simulink model "ElectricVehicleThermalManagementWithHeatPump_2026a_version"  (R2026a)
settings: Solver=VariableStepAuto  StopTime=3600  AbsTol=1e-3
PreLoadFcn:
  | init_nmpc
InitFcn:
  | init_nmpc
model workspace: external: MATLAB File ElectricVehicleThermalManagementWithHeatPumpParameters.m (data not in the file)
values from neighbouring files (symbols this model uses):
  battery_C1_LUT = [1913.6 12447 30609 ... (first row only)    [ElectricVehicleThermalManagementWithHeatPumpParameters.m]
  battery_capacity_LUT = [280.081 276.25 276.392]    [ElectricVehicleThermalManagementWithHeatPumpParameters.m]
  battery_cell_cp = 795    [ElectricVehicleThermalManagementWithHeatPumpParameters.m]
  battery_cell_mass = 2.5    [ElectricVehicleThermalManagementWithHeatPumpParameters.m]
  battery_Em_LUT = [3.4966 3.5057 3.5148 ... (first row only)    [ElectricVehicleThermalManagementWithHeatPumpParameters.m]
  battery_N_cells = 20    [ElectricVehicleThermalManagementWithHeatPumpParameters.m]
  battery_Qe_init = 0    [ElectricVehicleThermalManagementWithHeatPumpParameters.m]
  battery_R0_LUT = [0.0117 0.0085 0.009 ... (first row only)    [ElectricVehicleThermalManagementWithHeatPumpParameters.m]
  battery_R1_LUT = [0.0109 0.0029 0.0013 ... (first row only)    [ElectricVehicleThermalManagementWithHeatPumpParameters.m]
  battery_SOC_LUT = [0; 0.1; 0.25; 0.5; 0.75; 0.9; 1]    [ElectricVehicleThermalManagementWithHeatPumpParameters.m]
  battery_T_init = -5    [ElectricVehicleThermalManagementWithHeatPumpParameters.m]
  battery_temperature_LUT = [5 20 40]    [ElectricVehicleThermalManagementWithHeatPumpParameters.m]
  cabin_duct_area = 0.04    [ElectricVehicleThermalManagementWithHeatPumpParameters.m]
  cabin_T_init = -5    [ElectricVehicleThermalManagementWithHeatPumpParameters.m]
  chiller_area_primary = 0.43982297150257105    (= 0.439822971503)    [ElectricVehicleThermalManagementWithHeatPumpParameters.m]
  chiller_N_baffles = 3    [ElectricVehicleThermalManagementWithHeatPumpParameters.m]
  chiller_N_tubes = 100    [ElectricVehicleThermalManagementWithHeatPumpParameters.m]
  chiller_tube_D = 0.0035    [ElectricVehicleThermalManagementWithHeatPumpParameters.m]
  chiller_tube_L = 0.4    [ElectricVehicleThermalManagementWithHeatPumpParameters.m]
  chiller_wall_conductivity = 240    [ElectricVehicleThermalManagementWithHeatPumpParameters.m]
  chiller_wall_thickness = 0.0001    [ElectricVehicleThermalManagementWithHeatPumpParameters.m]
  cond_evap_air_area_flow = 0.3906    [ElectricVehicleThermalManagementWithHeatPumpParameters.m]
  cond_evap_air_area_primary = 1.4834999999999998    (= 1.4835)    [ElectricVehicleThermalManagementWithHeatPumpParameters.m]
  cond_evap_W = 0.015    [ElectricVehicleThermalManagementWithHeatPumpParameters.m]
  cond_evap_wall_conductivity = 240    [ElectricVehicleThermalManagementWithHeatPumpParameters.m]
  cond_evap_wall_thickness = 0.0001    [ElectricVehicleThermalManagementWithHeatPumpParameters.m]
  coolant_channel_D = 0.0092    [ElectricVehicleThermalManagementWithHeatPumpParameters.m]
  coolant_pipe_D = 0.019    [ElectricVehicleThermalManagementWithHeatPumpParameters.m]
  coolant_T_init = -5    [ElectricVehicleThermalManagementWithHeatPumpParameters.m]
  coolant_tank_area = 0.0121    [ElectricVehicleThermalManagementWithHeatPumpParameters.m]
  coolant_tank_volume = 1.25    [ElectricVehicleThermalManagementWithHeatPumpParameters.m]
  coolant_valve_D_ratio_max = 0.95    [ElectricVehicleThermalManagementWithHeatPumpParameters.m]
  coolant_valve_D_ratio_min = 0.001    [ElectricVehicleThermalManagementWithHeatPumpParameters.m]
  coolant_valve_displacement = 0.0063    [ElectricVehicleThermalManagementWithHeatPumpParameters.m]
  coolant_valve_S_max = 0.0053    [ElectricVehicleThermalManagementWithHeatPumpParameters.m]
  evaporator_air_area_flow = 0.12    [ElectricVehicleThermalManagementWithHeatPumpParameters.m]
  evaporator_air_area_primary = 0.4323    [ElectricVehicleThermalManagementWithHeatPumpParameters.m]
  evaporator_W = 0.015    [ElectricVehicleThermalManagementWithHeatPumpParameters.m]
  evaporator_wall_conductivity = 240    [ElectricVehicleThermalManagementWithHeatPumpParameters.m]
  evaporator_wall_thickness = 0.0001    [ElectricVehicleThermalManagementWithHeatPumpParameters.m]
  expansion_valve_D_ratio_max = 0.9    [ElectricVehicleThermalManagementWithHeatPumpParameters.m]
  hex_area_primary = 0.070371675440411369    (= 0.0703716754404)    [ElectricVehicleThermalManagementWithHeatPumpParameters.m]
  hex_N_tubes = 64    [ElectricVehicleThermalManagementWithHeatPumpParameters.m]
  hex_tube_D = 0.0035    [ElectricVehicleThermalManagementWithHeatPumpParameters.m]
  hex_wall_conductivity = 240    [ElectricVehicleThermalManagementWithHeatPumpParameters.m]
  hex_wall_thickness = 0.0001    [ElectricVehicleThermalManagementWithHeatPumpParameters.m]
  inner_cond_air_area_flow = 0.1953    [ElectricVehicleThermalManagementWithHeatPumpParameters.m]
  inner_cond_air_area_primary = 0.99520000000000008    (= 0.9952)    [ElectricVehicleThermalManagementWithHeatPumpParameters.m]
  inner_cond_W = 0.02    [ElectricVehicleThermalManagementWithHeatPumpParameters.m]
  inner_cond_wall_conductivity = 240    [ElectricVehicleThermalManagementWithHeatPumpParameters.m]
  inner_cond_wall_thickness = 0.0001    [ElectricVehicleThermalManagementWithHeatPumpParameters.m]
  pump_speed_max = 1000    [ElectricVehicleThermalManagementWithHeatPumpParameters.m]
  radiator_air_area_flow = 0.097499999999999989    (= 0.0975)    [ElectricVehicleThermalManagementWithHeatPumpParameters.m]
  radiator_air_area_primary = 0.43687499999999996    (= 0.436875)    [ElectricVehicleThermalManagementWithHeatPumpParameters.m]
  radiator_W = 0.015    [ElectricVehicleThermalManagementWithHeatPumpParameters.m]
  radiator_wall_conductivity = 240    [ElectricVehicleThermalManagementWithHeatPumpParameters.m]
  radiator_wall_thickness = 0.0001    [ElectricVehicleThermalManagementWithHeatPumpParameters.m]
  refrigerant_p_init = 0.25    [ElectricVehicleThermalManagementWithHeatPumpParameters.m]
  refrigerant_pipe_D = 0.01    [ElectricVehicleThermalManagementWithHeatPumpParameters.m]
  refrigerant_valve_D_ratio_max = 0.95    [ElectricVehicleThermalManagementWithHeatPumpParameters.m]
  refrigerant_valve_displacement = 0.005    [ElectricVehicleThermalManagementWithHeatPumpParameters.m]
libraries: fl_lib x227, nesl_utility x162, SimscapeFluids_lib x30, LiBatteryElements_lib x16, slpidlib x3, SignalEditorBlockLib x1
(part 9 of 13)

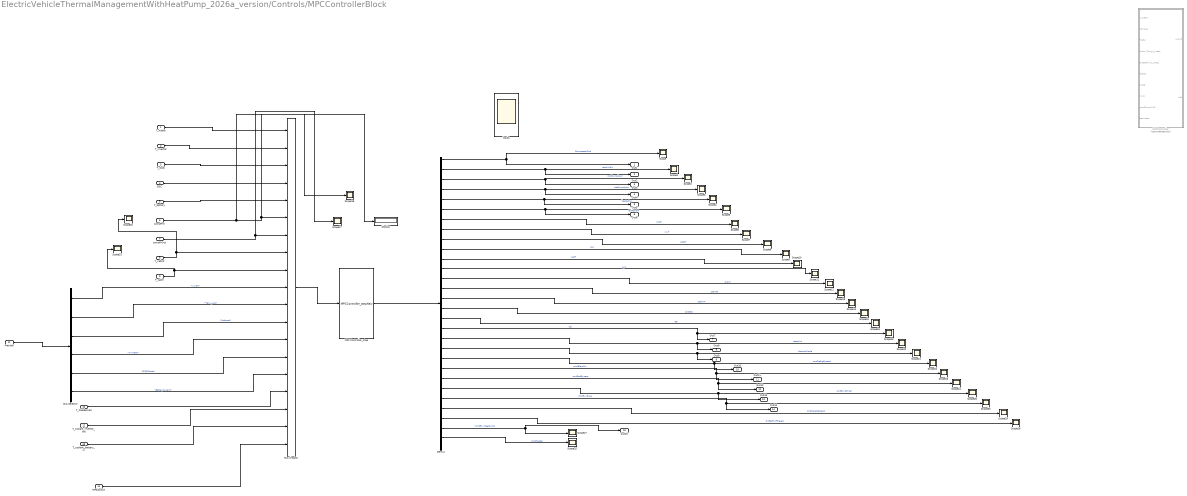
== system ElectricVehicleThermalManagementWithHeatPump_2026a_version/Controls/MPCControllerBlock ==
  T_motor : Inport
  T_inverter : Inport  Port=2
  T_dcdc : Inport  Port=3
  SOC : Inport  Port=4
  T_battery : Inport  Port=5
  compPrIn : Inport  Port=6
  compPrOut : Inport  Port=7
  T_cabInt : Inport  Port=8
  T_cabin : Inport  Port=9
  T_Cabdesired : Inport  Port=10
  Preview : Inport  Port=11
  T_coolant_inverter_out : Inport  Port=12
  T_coolant_battery_in : Inport  Port=13
  MPCSwitch : Inport  Port=14
  Bus Creator : BusCreator  Inputs=19
  Bus Selector : BusSelector  OutputSignals=v_vec,Tenv_vec,MotHeat,InvHeat,DCDCHeat,BatteryCurrent
  Demux : Demux  Outputs=30
  Display : Display
  "Inputs " : Scope
      settings: IsFloating=on  Floating=on  DataLoggingVariableName=ScopeData2
  MPC Controller_step : MATLABFcn  MATLABFcn=MPCController_stepNew  OutputDimensions=30
  MPCController : MATLAB Function  Commented=on  TreatAsAtomicUnit=on
  Scope{,1..32} (33 alike) : Scope
      Scope settings: ActiveDisplayYMinimum=2860.86724  ActiveDisplayYMaximum=6348.79253
      Scope1 settings: ActiveDisplayYMinimum=-0.01483  ActiveDisplayYMaximum=0.16831  DataLoggingVariableName=ScopeData4
      Scope10 settings: ActiveDisplayYMinimum=288.13418  ActiveDisplayYMaximum=288.13679  DataLoggingVariableName=ScopeData13
      Scope11 settings: ActiveDisplayYMinimum=-122277.20215  ActiveDisplayYMaximum=1.60049481934E+6
      Scope12 settings: ActiveDisplayYMinimum=-135086.04367  ActiveDisplayYMaximum=3.52084504555E+6  DataLoggingVariableName=ScopeData15
      Scope13 settings: ActiveDisplayYMinimum=287.60244  ActiveDisplayYMaximum=292.90804  DataLoggingVariableName=ScopeData16
      Scope14 settings: ActiveDisplayYMinimum=263.5349  ActiveDisplayYMaximum=264.17335  DataLoggingVariableName=ScopeData17
      Scope15 settings: ActiveDisplayYMinimum=-0.125  ActiveDisplayYMaximum=1.125  DataLoggingVariableName=ScopeData18
      Scope16 settings: ActiveDisplayYMinimum=-62.25  ActiveDisplayYMaximum=850.25  DataLoggingVariableName=ScopeData19
      Scope17 settings: ActiveDisplayYMinimum=-0.22381  ActiveDisplayYMaximum=4.01427  DataLoggingVariableName=ScopeData21
      Scope18 settings: ActiveDisplayYMinimum=0.12091  ActiveDisplayYMaximum=0.20879  DataLoggingVariableName=ScopeData22
      Scope19 settings: ActiveDisplayYMinimum=6.82463350048E+6  ActiveDisplayYMaximum=3.038905731081E+7
      Scope2 settings: ActiveDisplayYMinimum=9.75705  ActiveDisplayYMaximum=912.18659  DataLoggingVariableName=ScopeData5
      Scope20 settings: ActiveDisplayYMinimum=1  ActiveDisplayYMaximum=3  DataLoggingVariableName=ScopeData2
      Scope21 settings: ActiveDisplayYMinimum=1  ActiveDisplayYMaximum=3  DataLoggingVariableName=ScopeData3
      Scope22 settings: ActiveDisplayYMinimum=0.9  ActiveDisplayYMaximum=1.1  DataLoggingVariableName=ScopeData4
      Scope23 settings: ActiveDisplayYMinimum=3.2105763177086E+8  ActiveDisplayYMaximum=8.150914987049E+8  DataLoggingVariableName=ScopeData5
      Scope24 settings: ActiveDisplayYMinimum=0.9  ActiveDisplayYMaximum=1.1  DataLoggingVariableName=ScopeData6
      Scope25 settings: ActiveDisplayYMinimum=-1  ActiveDisplayYMaximum=1  DataLoggingVariableName=ScopeData7
      Scope26 settings: ActiveDisplayYMinimum=-1  ActiveDisplayYMaximum=1  DataLoggingVariableName=ScopeData8
      Scope27 settings: ActiveDisplayYMinimum=0.9  ActiveDisplayYMaximum=1.1  DataLoggingVariableName=ScopeData9
      Scope28 settings: ActiveDisplayYMinimum=3.2105763177086E+8  ActiveDisplayYMaximum=8.150914987049E+8  DataLoggingVariableName=ScopeData10
      Scope29 settings: ActiveDisplayYMinimum=0.9  ActiveDisplayYMaximum=1.1  DataLoggingVariableName=ScopeData11
      Scope3 settings: ActiveDisplayYMinimum=9.75705  ActiveDisplayYMaximum=912.18659  DataLoggingVariableName=ScopeData6
      Scope30 settings: ActiveDisplayYMinimum=-1  ActiveDisplayYMaximum=1  DataLoggingVariableName=ScopeData12
      Scope31 settings: ActiveDisplayYMinimum=-0.22381  ActiveDisplayYMaximum=4.01427
      Scope32 settings: ActiveDisplayYMinimum=-0.22381  ActiveDisplayYMaximum=4.01427  DataLoggingVariableName=ScopeData2
      Scope4 settings: ActiveDisplayYMinimum=749.75794  ActiveDisplayYMaximum=3630.06102  DataLoggingVariableName=ScopeData7
      Scope5 settings: ActiveDisplayYMinimum=-121.45882  ActiveDisplayYMaximum=1093.12937  DataLoggingVariableName=ScopeData8
      Scope6 settings: ActiveDisplayYMinimum=283.13748  ActiveDisplayYMaximum=283.14002  DataLoggingVariableName=ScopeData9
      Scope7 settings: ActiveDisplayYMinimum=279.17711  ActiveDisplayYMaximum=319.38081  DataLoggingVariableName=ScopeData10
      Scope8 settings: ActiveDisplayYMinimum=283.13677  ActiveDisplayYMaximum=283.14932  DataLoggingVariableName=ScopeData11
      Scope9 settings: ActiveDisplayYMinimum=0.96023  ActiveDisplayYMaximum=1.00439  DataLoggingVariableName=ScopeData12
  Out1 : Outport
  Out2 : Outport  Port=2
  Out3 : Outport  Port=3
  Out4 : Outport  Port=4
  Out5 : Outport  Port=5
  Out6 : Outport  Port=6
  Out7 : Outport  Port=7
  Out8 : Outport  Port=8
  Out9 : Outport  Port=9
  Out10 : Outport  Port=10
  Out11 : Outport  Port=11
  Out12 : Outport  Port=12
  Out13 : Outport  Port=13
  Out14 : Outport  Port=14
  Out15 : Outport  Port=15
  wires:
  Bus Creator/1 -> MPC Controller_step/1
  T_Cabdesired/1 -> Bus Creator/16
  Preview/1 -> Bus Selector/1
  Bus Selector/2 -> Bus Creator/11  "<Tenv_vec>"
  Bus Selector/3 -> Bus Creator/12  "<MotHeat>"
  Bus Selector/4 -> Bus Creator/13  "<InvHeat>"
  Bus Selector/5 -> Bus Creator/14  "<DCDCHeat>"
  Bus Selector/6 -> Bus Creator/15  "<BatteryCurrent>"
  T_coolant_inverter_out/1 -> Bus Creator/17
  T_coolant_battery_in/1 -> Bus Creator/18
  T_motor/1 -> Bus Creator/1
  T_inverter/1 -> Bus Creator/2
  T_dcdc/1 -> Bus Creator/3
  SOC/1 -> Bus Creator/4
  T_battery/1 -> Bus Creator/5
  compPrIn/1 -> Scope18/1, Display/1, Bus Creator/6
  compPrOut/1 -> Scope17/1, Bus Creator/7
  T_cabInt/1 -> Scope32/1, Bus Creator/8
  T_cabin/1 -> Scope31/1, Bus Creator/9
  MPC Controller_step/1 -> Demux/1
  Demux/1 -> Out1/1, Scope/1  "CompressorSpd"
  Demux/2 -> Out2/1, Scope1/1  "cabAirMfIn"
  Demux/3 -> Out3/1, Scope2/1  "motPumpNrpm"
  Demux/4 -> Out4/1, Scope3/1  "batPumpNrpm"
  Demux/5 -> Out5/1, Scope4/1  "heaterPwr"
  Demux/6 -> Out6/1, Scope5/1  "radFanrpm"
  Demux/7 -> Scope6/1  "motT"
  Demux/8 -> Scope7/1  "invT"
  Demux/9 -> Scope8/1  "dcdcT"
  Demux/10 -> Scope9/1  "soc"
  Demux/11 -> Scope10/1  "batT"
  Demux/12 -> Scope11/1  "p_in"
  Demux/13 -> Scope12/1  "p_out"
  Demux/14 -> Scope13/1  "cabIntT"
  Demux/15 -> Scope14/1  "cabAirT"
  Demux/16 -> Scope15/1  "success"
  Demux/17 -> Scope16/1  "iter"
  Demux/18 -> Out7/1, Scope19/1  "obj"
  Demux/19 -> Out8/1, Scope20/1  "setpoint"
  Demux/20 -> Out9/1, Scope21/1  "thermalMode"
  Demux/21 -> Out10/1, Scope22/1  "cmdRefrigBypass"
  Demux/22 -> Out11/1, Scope23/1  "cmdBlendAir"
  Demux/23 -> Out12/1, Scope24/1  "cmdRadBypass"
  Demux/24 -> Out13/1, Scope26/1  "cmdExvChiller"
  Demux/29 -> Scope25/1  "cmdHeater"
  Demux/28 -> Scope27/1, Out15/1  "<cmdExvHeatpump"
  Demux/27 -> Scope28/1  "clntBatTinFiltered"
  Demux/26 -> Scope29/1  "cmdParallelSerial"
  Demux/25 -> Out14/1, Scope30/1  "cmdExvEvap"
  Bus Selector/1 -> Bus Creator/10  "<v_vec>"
  MPCSwitch/1 -> Bus Creator/19
